simulink model "banc_moteur_A2212"  (R2025b)
settings: Solver=ode45  StartTime=0.0  StopTime=inf  MaxStep=5e-4  RelTol=1e-4
InitFcn:
  | % Charge les paramètres s'ils ne sont pas encore dans l'espace de travail
  | if ~exist('Jm', 'var') || ~exist('port_esp32', 'var'), run(fullfile(fileparts(get_param(bdroot, 'FileName')), 'banc_parametres.m')); end
values from neighbouring files (symbols this model uses):
  a0 = -(Kt*Ke/(Jm*Rm) + fv/Jm)    (= -3.62456229571)    [banc_parametres.m]
  A_eso = Aa - L*Ca    [banc_parametres.m]
  b0 = Kt/(Jm*Rm)    (= 526.858905372)    [banc_parametres.m]
  B_eso = [Ba L]    [banc_parametres.m]
  bruit_actif = 0    [banc_parametres.m]
  eso_actif = 1    [banc_parametres.m]
  fv = 5e-6    (= 5e-06)    [banc_parametres.m]
  imp_banc_max = 1700    [banc_parametres.m]
  imp_banc_min = 1300    [banc_parametres.m]
  imp_course = 500    [banc_parametres.m]
  imp_neutre = 1500    [banc_parametres.m]
  Jm = J_rotor + J_disque + J_vis    (= 0.00016183)    [banc_parametres.m]
  K = 8    [banc_parametres.m]
  Ke = 60/(2*pi*KV)    (= 0.00682092613251)    [banc_parametres.m]
  Kt = Ke    (= 0.00682092613251)    [banc_parametres.m]
  Lm = 30e-6    (= 3e-05)    [banc_parametres.m]
  perturbation_active = 0    [banc_parametres.m]
  Rm = 0.08    [banc_parametres.m]
  sigma_bruit = 2    [banc_parametres.m]
  t_pert = 3    [banc_parametres.m]
  tau_L = 0.03    [banc_parametres.m]
  Ts_bruit = 0.005    [banc_parametres.m]
  Ts_com = 0.01    [banc_parametres.m]
  Vbat = 11.1    [banc_parametres.m]
  Vmax = Vbat    (= 11.1)    [banc_parametres.m]
  w_amp = 100    [banc_parametres.m]
  w_moy = 300    [banc_parametres.m]
  w_puls = 0.5    [banc_parametres.m]
libraries: instrumentseriallib x3, simulink x2
settings Model: Creator=FOFIEVIGOLBRYAN  LastModifiedBy=FOFIEVIGOLBRYAN

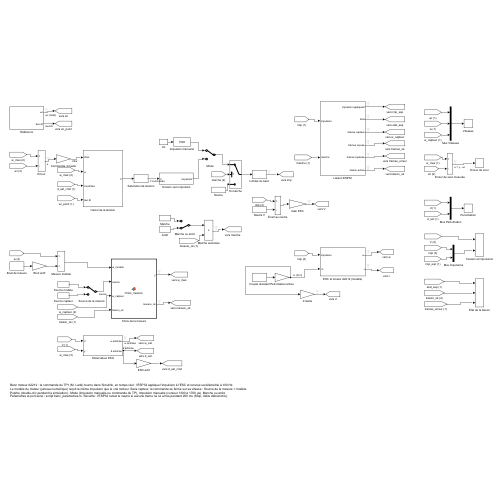
[thumbnail: Simulink's stored preview of the top-level diagram]
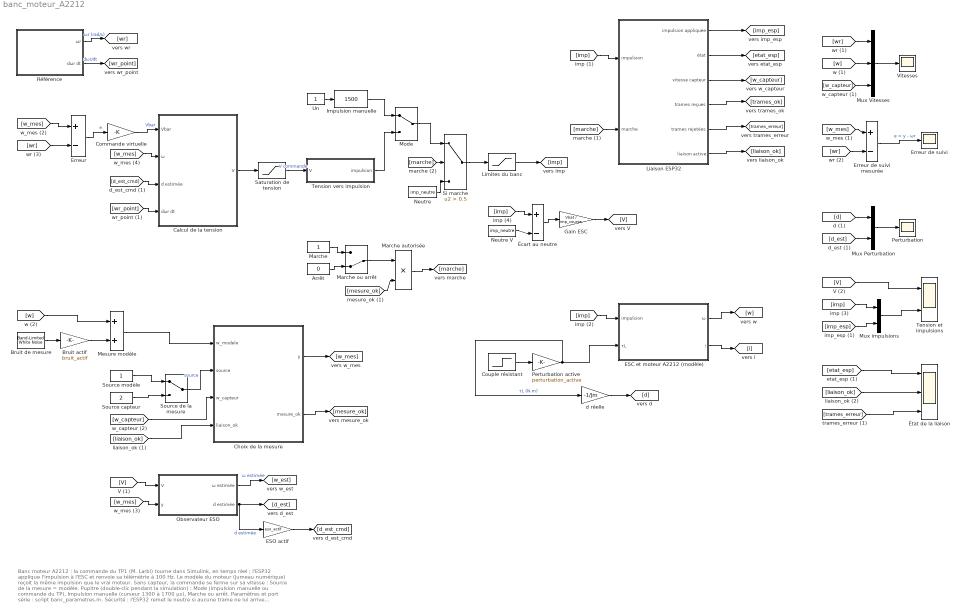
== system banc_moteur_A2212 ==
  note: Banc moteur A2212 : la commande du TP1 (M. Larbi) tourne dans Simulink, en temps réel ; l'ESP32 applique l'impulsion à l'ESC et renvoie sa télémétrie à 100 Hz.
      | Le modèle du moteur (jumeau numérique) reçoit la même impulsion que le vrai moteur. Sans capteur, la commande se ferme sur sa vitesse : Source de la mesure = modèle.
      | Pupitre (double-clic pendant la simulation) : Mode (impulsion manuelle ou commande du TP), Impulsion manuelle (curseur 1300 à 1700 µs), Marche ou arrêt.
      | Paramètres et port série : script banc_parametres.m. Sécurité : l'ESP32 remet le neutre si aucune trame ne lui arrive pendant 200 ms (Stop, câble débranché).
  Arrêt : Constant  Value=0
  Bruit actif : Gain  Gain=bruit_actif
  Bruit de mesure : simulink/Sources/Band-Limited White Noise  Cov=sigma_bruit^2 * Ts_bruit  Ts=Ts_bruit  seed=23341
  Calcul de la tension : Subsystem
  Choix de la mesure : MATLAB Function  TreatAsAtomicUnit=on
  Commande virtuelle : Gain  Gain=-K
  Couple résistant : Step  Time=t_pert  After=tau_L  SampleTime=0
  ESC et moteur A2212 (modèle) : Subsystem
  ESO actif : Gain  Gain=eso_actif
  Erreur : Sum  Inputs=+-
  Erreur de suivi : Scope
  Erreur de suivi mesurée : Sum  Inputs=+-
  Gain ESC : Gain  Gain=Vbat / imp_course
  Impulsion manuelle : simulink/Math Operations/Slider Gain  gain=1500  low=1300  high=1700
  Liaison ESP32 : Subsystem
  Limites du banc : Saturate  UpperLimit=imp_banc_max  LowerLimit=imp_banc_min
  Marche : Constant
  Marche autorisée : Product
  Marche ou arrêt : ManualSwitch  CurrentSetting=0
  Mesure modèle : Sum
  Mode : ManualSwitch
  Mux Perturbation : Mux  Inputs=2
  Mux Vitesses : Mux  Inputs=3
  Mux impulsions : Mux  Inputs=2
  Neutre : Constant  Value=imp_neutre
  Neutre V : Constant  Value=imp_neutre
  Observateur ESO : Subsystem
  Perturbation : Scope
  Perturbation active : Gain  Gain=perturbation_active
  Référence : Subsystem
  Saturation de tension : Saturate  UpperLimit=Vmax  LowerLimit=-Vmax
  Si marche : Switch  Criteria=u2 > Threshold  Threshold=0.5  SaturateOnIntegerOverflow=off  InputSameDT=off
  Source capteur : Constant  Value=2
  Source de la mesure : ManualSwitch
  Source modèle : Constant
  Tension et impulsions : Scope  NumInputPorts=2
      settings: Title=Impulsion envoyée et appliquée (µs)
  Tension vers impulsion : Subsystem
  Un : Constant
  Vitesses : Scope
  d réelle : Gain  Gain=-1/Jm
  Écart au neutre : Sum  Inputs=+-
  État de la liaison : Scope  NumInputPorts=3
      settings: ActiveDisplayString=3  Title=Trames rejetées
  wires:
  Référence/1(ωr) -> [wr]  "ωr (rad/s)"
  Référence/2(dωr dt) -> [wr_point]  "dωr/dt"
  [w_mes] -> Erreur/1
  [wr] -> Erreur/2
  Erreur/1 -> Commande virtuelle/1  "e"
  Commande virtuelle/1 -> Calcul de la tension/1(Vbar)  "Vbar"
  [w_mes] -> Calcul de la tension/2(ω)
  [d_est_cmd] -> Calcul de la tension/3(d estimée)
  [wr_point] -> Calcul de la tension/4(dωr dt)
  Calcul de la tension/1(V) -> Saturation de tension/1
  Saturation de tension/1 -> Tension vers impulsion/1(V)  "V commande"
  Un/1 -> Impulsion manuelle/1
  Impulsion manuelle/1 -> Mode/1
  Tension vers impulsion/1(impulsion) -> Mode/2
  Marche/1 -> Marche ou arrêt/1
  Arrêt/1 -> Marche ou arrêt/2
  Marche ou arrêt/1 -> Marche autorisée/1
  [mesure_ok] -> Marche autorisée/2
  Marche autorisée/1 -> [marche]
  Mode/1 -> Si marche/1
  [marche] -> Si marche/2
  Neutre/1 -> Si marche/3
  Si marche/1 -> Limites du banc/1
  Limites du banc/1 -> [imp]
  [imp] -> Écart au neutre/1
  Neutre V/1 -> Écart au neutre/2
  Écart au neutre/1 -> Gain ESC/1
  Gain ESC/1 -> [V]
  [imp] -> Liaison ESP32/1(impulsion)
  [marche] -> Liaison ESP32/2(marche)
  Liaison ESP32/1(impulsion appliquée) -> [imp_esp]
  Liaison ESP32/2(état) -> [etat_esp]
  Liaison ESP32/3(vitesse capteur) -> [w_capteur]
  Liaison ESP32/4(trames reçues) -> [trames_ok]
  Liaison ESP32/5(trames rejetées) -> [trames_erreur]
  Liaison ESP32/6(liaison active) -> [liaison_ok]
  [imp] -> ESC et moteur A2212 (modèle)/1(impulsion)
  Couple résistant/1 -> Perturbation active/1
  Perturbation active/1 -> ESC et moteur A2212 (modèle)/2(τL), d réelle/1  "τL (N.m)"
  d réelle/1 -> [d]
  ESC et moteur A2212 (modèle)/1(ω) -> [w]
  ESC et moteur A2212 (modèle)/2(i) -> [i]
  Bruit de mesure/1 -> Bruit actif/1
  [w] -> Mesure modèle/1
  Bruit actif/1 -> Mesure modèle/2
  Source modèle/1 -> Source de la mesure/1
  Source capteur/1 -> Source de la mesure/2
  Mesure modèle/1 -> Choix de la mesure/1(w_modele)
  Source de la mesure/1 -> Choix de la mesure/2(source)  "source"
  [w_capteur] -> Choix de la mesure/3(w_capteur)
  [liaison_ok] -> Choix de la mesure/4(liaison_ok)
  Choix de la mesure/1(y) -> [w_mes]
  Choix de la mesure/2(mesure_ok) -> [mesure_ok]
  [V] -> Observateur ESO/1(V)
  [w_mes] -> Observateur ESO/2(y)
  Observateur ESO/1(ω estimée) -> [w_est]  "ω estimée"
  Observateur ESO/2(d estimée) -> [d_est], ESO actif/1  "d estimée"
  ESO actif/1 -> [d_est_cmd]
  Mux Vitesses/1 -> Vitesses/1
  [wr] -> Mux Vitesses/1
  [w] -> Mux Vitesses/2
  [w_capteur] -> Mux Vitesses/3
  Mux Perturbation/1 -> Perturbation/1
  [d] -> Mux Perturbation/1
  [d_est] -> Mux Perturbation/2
  [V] -> Tension et impulsions/1
  [imp] -> Mux impulsions/1
  [imp_esp] -> Mux impulsions/2
  Mux impulsions/1 -> Tension et impulsions/2
  [etat_esp] -> État de la liaison/1
  [liaison_ok] -> État de la liaison/2
  [trames_erreur] -> État de la liaison/3
  [w_mes] -> Erreur de suivi mesurée/1
  [wr] -> Erreur de suivi mesurée/2
  Erreur de suivi mesurée/1 -> Erreur de suivi/1  "e = y - ωr"

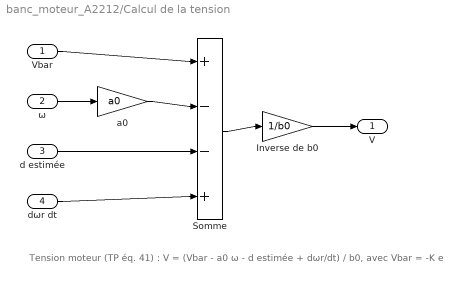
== system banc_moteur_A2212/Calcul de la tension ==
  note: Tension moteur (TP éq. 41) : V = (Vbar - a0 ω - d estimée + dωr/dt) / b0, avec Vbar = -K e
  Vbar : Inport
  ω : Inport  Port=2
  d estimée : Inport  Port=3
  dωr dt : Inport  Port=4
  Inverse de b0 : Gain  Gain=1/b0
  Somme : Sum  Inputs=+--+
  a0 : Gain  Gain=a0
  V : Outport
  wires:
  Vbar/1 -> Somme/1
  ω/1 -> a0/1
  a0/1 -> Somme/2
  d estimée/1 -> Somme/3
  dωr dt/1 -> Somme/4
  Somme/1 -> Inverse de b0/1
  Inverse de b0/1 -> V/1

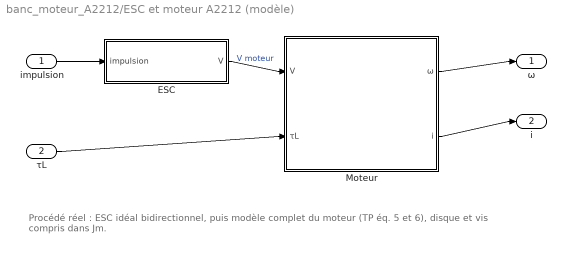
== system banc_moteur_A2212/ESC et moteur A2212 (modèle) ==
  note: Procédé réel : ESC idéal bidirectionnel, puis modèle complet du moteur (TP éq. 5 et 6), disque et vis compris dans Jm.
  impulsion : Inport
  τL : Inport  Port=2
  ESC : Subsystem
  Moteur : Subsystem
  ω : Outport
  i : Outport  Port=2
  wires:
  impulsion/1 -> ESC/1(impulsion)
  ESC/1(V) -> Moteur/1(V)  "V moteur"
  τL/1 -> Moteur/2(τL)
  Moteur/1(ω) -> ω/1
  Moteur/2(i) -> i/1

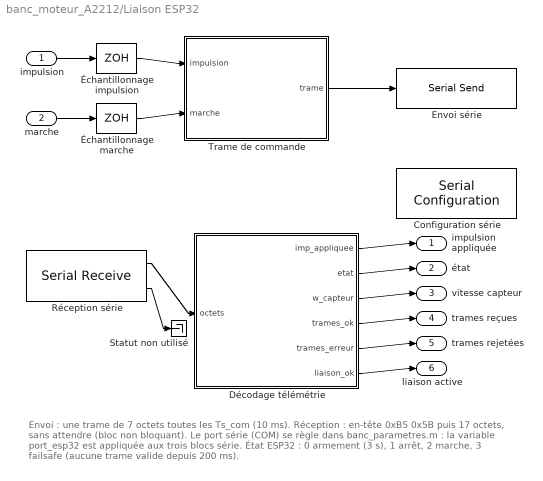
== system banc_moteur_A2212/Liaison ESP32 ==
  note: Envoi : une trame de 7 octets toutes les Ts_com (10 ms). Réception : en-tête 0xB5 0x5B puis 17 octets, sans attendre (bloc non bloquant).
      | Le port série (COM) se règle dans banc_parametres.m : la variable port_esp32 est appliquée aux trois blocs série.
      | État ESP32 : 0 armement (3 s), 1 arrêt, 2 marche, 3 failsafe (aucune trame valide depuis 200 ms).
  impulsion : Inport
  marche : Inport  Port=2
  Configuration série : instrumentseriallib/Serial Configuration  Priority=-200000  PortSel=COM3  Port=COM3  ComPort=COM3  BaudRate=115200  DataBits=8  Parity=none  StopBits=1  ByteOrder=little-endian  FlowControl=none  Timeout=1  SimulateUsing=Interpreted execution  BlockInModel=on  aMode=1
  Décodage télémétrie : MATLAB Function  TreatAsAtomicUnit=on
  Envoi série : instrumentseriallib/Serial Send  Priority=1  PortSel=COM3  Port=COM3  ComPort=COM3  Header=[]  Terminator=<none>  CustomTerminator=[]  EnableBlockingMode=off  SimulateUsing=Interpreted execution  BlockInModel=on  aMode=1
  Réception série : instrumentseriallib/Serial Receive  Priority=1  PortSel=COM3  Port=COM3  ComPort=COM3  DataType=uint8  SaveDataType=uint8  ToggleHeader=on  Header=[181 91]  ToggleDataSize=on  DataSize=[17 1]  ToggleTerminator=off  Terminator=<none>  CustomTerminator=[]  InputFormat=Column major  EnableBlockingMode=off  ActionDataUnavailable=Output last received value  ActionWhenDataUnavailable=Output last received value  CustomValue=0  SampleTime=Ts_com  SimulateUsing=Interpreted execution  BlockInModel=on  aMode=1  LibraryInUse=instrumentlib
  Statut non utilisé : Terminator
  Trame de commande : MATLAB Function  TreatAsAtomicUnit=on
  Échantillonnage impulsion : ZeroOrderHold  SampleTime=Ts_com
  Échantillonnage marche : ZeroOrderHold  SampleTime=Ts_com
  impulsion appliquée : Outport
  état : Outport  Port=2
  vitesse capteur : Outport  Port=3
  trames reçues : Outport  Port=4
  trames rejetées : Outport  Port=5
  liaison active : Outport  Port=6
  wires:
  impulsion/1 -> Échantillonnage impulsion/1
  marche/1 -> Échantillonnage marche/1
  Échantillonnage impulsion/1 -> Trame de commande/1(impulsion)
  Échantillonnage marche/1 -> Trame de commande/2(marche)
  Trame de commande/1(trame) -> Envoi série/1
  Réception série/1 -> Décodage télémétrie/1(octets)
  Réception série/2 -> Statut non utilisé/1
  Décodage télémétrie/1(imp_appliquee) -> impulsion appliquée/1
  Décodage télémétrie/2(etat) -> état/1
  Décodage télémétrie/3(w_capteur) -> vitesse capteur/1
  Décodage télémétrie/4(trames_ok) -> trames reçues/1
  Décodage télémétrie/5(trames_erreur) -> trames rejetées/1
  Décodage télémétrie/6(liaison_ok) -> liaison active/1

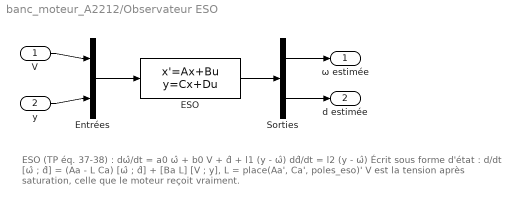
== system banc_moteur_A2212/Observateur ESO ==
  note: ESO (TP éq. 37-38) :  dω̂/dt = a0 ω̂ + b0 V + d̂ + l1 (y - ω̂)     dd̂/dt = l2 (y - ω̂)
      | Écrit sous forme d'état :  d/dt [ω̂ ; d̂] = (Aa - L Ca) [ω̂ ; d̂] + [Ba  L] [V ; y],  L = place(Aa', Ca', poles_eso)'
      | V est la tension après saturation, celle que le moteur reçoit vraiment.
  V : Inport
  y : Inport  Port=2
  ESO : StateSpace  A=A_eso  B=B_eso  C=eye(2)  D=zeros(2)  InitialCondition=[0; 0]
  Entrées : Mux  Inputs=2
  Sorties : Demux  Outputs=2
  ω estimée : Outport
  d estimée : Outport  Port=2
  wires:
  V/1 -> Entrées/1
  y/1 -> Entrées/2
  Entrées/1 -> ESO/1
  ESO/1 -> Sorties/1
  Sorties/1 -> ω estimée/1
  Sorties/2 -> d estimée/1

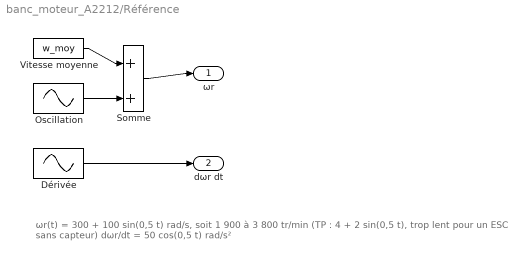
== system banc_moteur_A2212/Référence ==
  note: ωr(t) = 300 + 100 sin(0,5 t) rad/s, soit 1 900 à 3 800 tr/min (TP : 4 + 2 sin(0,5 t), trop lent pour un ESC sans capteur)
      | dωr/dt = 50 cos(0,5 t) rad/s²
  Dérivée : Sin  Amplitude=w_amp * w_puls  Frequency=w_puls  Phase=pi/2  SampleTime=0
  Oscillation : Sin  Amplitude=w_amp  Frequency=w_puls  SampleTime=0
  Somme : Sum
  Vitesse moyenne : Constant  Value=w_moy
  ωr : Outport
  dωr dt : Outport  Port=2
  wires:
  Vitesse moyenne/1 -> Somme/1
  Oscillation/1 -> Somme/2
  Somme/1 -> ωr/1
  Dérivée/1 -> dωr dt/1

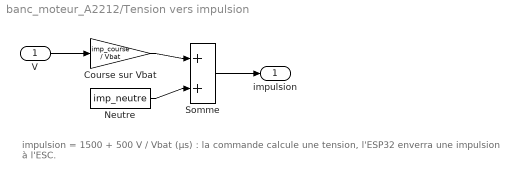
== system banc_moteur_A2212/Tension vers impulsion ==
  note: impulsion = 1500 + 500 V / Vbat (µs) : la commande calcule une tension, l'ESP32 enverra une impulsion à l'ESC.
  V : Inport
  Course sur Vbat : Gain  Gain=imp_course / Vbat
  Neutre : Constant  Value=imp_neutre
  Somme : Sum
  impulsion : Outport
  wires:
  V/1 -> Course sur Vbat/1
  Course sur Vbat/1 -> Somme/1
  Neutre/1 -> Somme/2
  Somme/1 -> impulsion/1

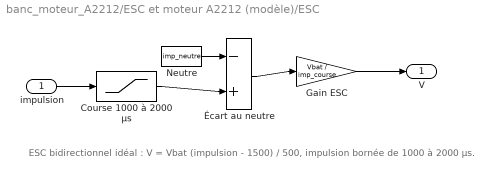
== system banc_moteur_A2212/ESC et moteur A2212 (modèle)/ESC ==
  note: ESC bidirectionnel idéal : V = Vbat (impulsion - 1500) / 500, impulsion bornée de 1000 à 2000 µs.
  impulsion : Inport
  Course 1000 à 2000 µs : Saturate  UpperLimit=imp_neutre + imp_course  LowerLimit=imp_neutre - imp_course
  Gain ESC : Gain  Gain=Vbat / imp_course
  Neutre : Constant  Value=imp_neutre
  Écart au neutre : Sum  Inputs=-+
  V : Outport
  wires:
  impulsion/1 -> Course 1000 à 2000 µs/1
  Neutre/1 -> Écart au neutre/1
  Course 1000 à 2000 µs/1 -> Écart au neutre/2
  Écart au neutre/1 -> Gain ESC/1
  Gain ESC/1 -> V/1

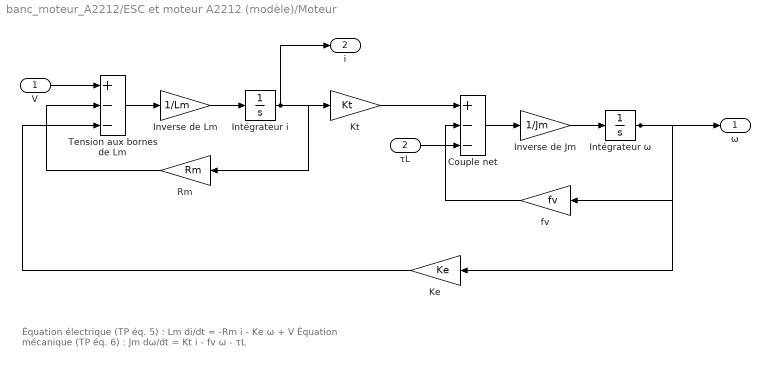
== system banc_moteur_A2212/ESC et moteur A2212 (modèle)/Moteur ==
  note: Équation électrique (TP éq. 5) :   Lm di/dt = -Rm i - Ke ω + V
      | Équation mécanique (TP éq. 6) :   Jm dω/dt = Kt i - fv ω - τL
  V : Inport
  τL : Inport  Port=2
  Couple net : Sum  Inputs=+--
  Intégrateur i : Integrator
  Intégrateur ω : Integrator
  Inverse de Jm : Gain  Gain=1/Jm
  Inverse de Lm : Gain  Gain=1/Lm
  Ke : Gain  Gain=Ke
  Kt : Gain  Gain=Kt
  Rm : Gain  Gain=Rm
  Tension aux bornes de Lm : Sum  Inputs=+--
  fv : Gain  Gain=fv
  ω : Outport
  i : Outport  Port=2
  wires:
  V/1 -> Tension aux bornes de Lm/1
  Tension aux bornes de Lm/1 -> Inverse de Lm/1
  Inverse de Lm/1 -> Intégrateur i/1
  Intégrateur i/1 -> Kt/1, Rm/1, i/1
  Rm/1 -> Tension aux bornes de Lm/2
  Kt/1 -> Couple net/1
  Couple net/1 -> Inverse de Jm/1
  Inverse de Jm/1 -> Intégrateur ω/1
  Intégrateur ω/1 -> ω/1, fv/1, Ke/1
  fv/1 -> Couple net/2
  τL/1 -> Couple net/3
  Ke/1 -> Tension aux bornes de Lm/3

== matlab function banc_moteur_A2212/Liaison ESP32/Décodage télémétrie ==
  data: octets input uint8 size=[17 1]; imp_appliquee output; etat output; w_capteur output; trames_ok output; trames_erreur output; liaison_ok output
function [imp_appliquee, etat, w_capteur, trames_ok, trames_erreur, liaison_ok] = decoder_telemetrie(octets)
% Trame ESP32 -> PC : 0xB5 0x5B | t_ms (uint32) | impulsion (uint16) | état (uint8) | seq (uint8)
%                     | vitesse (single, NaN sans capteur) | trames ok (uint16) | trames rejetées (uint16) | somme
% liaison_ok passe à 0 si la somme est fausse ou si le temps de l'ESP32 n'avance plus depuis 20 lectures (200 ms).
persistent t_prec n_fige
if isempty(t_prec), t_prec = -1; n_fige = 0; end
o = uint8(octets(:)).';
t_ms = double(typecast(o(1:4), 'uint32'));
valide = mod(sum(double(o(1:16))), 256) == double(o(17)) && t_ms > 0;   % que des zéros = rien reçu
if valide && t_ms ~= t_prec, n_fige = 0; else, n_fige = n_fige + 1; end
t_prec = t_ms;
liaison_ok = double(valide && n_fige < 20);
imp_appliquee = double(typecast(o(5:6), 'uint16'));
etat = double(o(7));
w_capteur = double(typecast(o(9:12), 'single'));
trames_ok = double(typecast(o(13:14), 'uint16'));
trames_erreur = double(typecast(o(15:16), 'uint16'));
if ~liaison_ok, w_capteur = NaN; end

== matlab function banc_moteur_A2212/Liaison ESP32/Trame de commande ==
  data: impulsion input; trame output; marche input
function trame = trame_commande(impulsion, marche)
% Trame PC -> ESP32 (7 octets) : 0xA5 0x5A | impulsion (uint16, petit-boutiste) | drapeaux | seq | somme
persistent seq
if isempty(seq), seq = 0; end
seq = mod(seq + 1, 256);
if ~isfinite(impulsion), impulsion = 1500; marche = 0; end   % jamais de NaN vers l'ESC
imp = round(min(max(impulsion, 1000), 2000));
lo = mod(imp, 256);
hi = floor(imp / 256);
drapeaux = double(marche > 0.5);
somme = mod(lo + hi + drapeaux + seq, 256);
trame = uint8([165; 90; lo; hi; drapeaux; seq; somme]);

== matlab function banc_moteur_A2212/Choix de la mesure ==
  data: w_modele input; y output; source input; w_capteur input; liaison_ok input; mesure_ok output
function [y, mesure_ok] = choix_mesure(w_modele, source, w_capteur, liaison_ok)
% source 1 : vitesse du modèle (aucun capteur monté) ; source 2 : vitesse mesurée par l'ESP32.
% Avec la source 2, si la liaison est coupée ou si le capteur ne donne rien (NaN), mesure_ok = 0
% et la marche est refusée : la commande ne doit jamais tourner sur une mesure absente.
y = w_modele;
mesure_ok = 1;
if source > 1.5
    if liaison_ok > 0.5 && isfinite(w_capteur)
        y = w_capteur;
    else
        mesure_ok = 0;
    end
end
